simulink model "multirotor_gn_model"  (R2025b)
settings: Solver=ode3  StartTime=0.0  StopTime=600  FixedStep=simulationSampleTime  RelTol=1e-3
values from neighbouring files (symbols this model uses):
  guidanceParams = [cfg.guidance.acceptanceRadiusM;      cfg.flight.transitSpeedMps; cfg.flight.searchSpeedMps;      cfg.flight.climbSpeedMps; cfg.flight.descentSpeedMps;      cfg.guidance.slowdownRadiusM;      cfg.guidance.landingHorizontalToleranceM;      cfg.guidance.landingAltitudeToleranceM]    [run_multirotor_mission.m]
  navigationFilterCoefficient = cfg.navigation.filterCoefficient    [run_multirotor_mission.m]
  navigationNoiseSeeds = mod(round(cfg.randomSeed)+(1:3)'*997,2^31-1)    [run_multirotor_mission.m]
  navigationNoiseVariance = cfg.navigation.positionNoiseStdM^2    [run_multirotor_mission.m]
  routeCount = mission.routeCount    [run_multirotor_mission.m]
  routePhasePadded = zeros(cfg.simulation.maxWaypoints,1)    [run_multirotor_mission.m]
  routeWaypointsPadded = zeros(cfg.simulation.maxWaypoints,3)    [run_multirotor_mission.m]
  simulationSampleTime = cfg.simulation.sampleTimeSec    [run_multirotor_mission.m]
  vehicleTimeConstantSec = cfg.vehicle.velocityTimeConstantSec    [run_multirotor_mission.m]
libraries: simulink x1
settings Model: Creator=andrei  LastModifiedBy=andrei
settings DataIOCC: SignalLogging=off

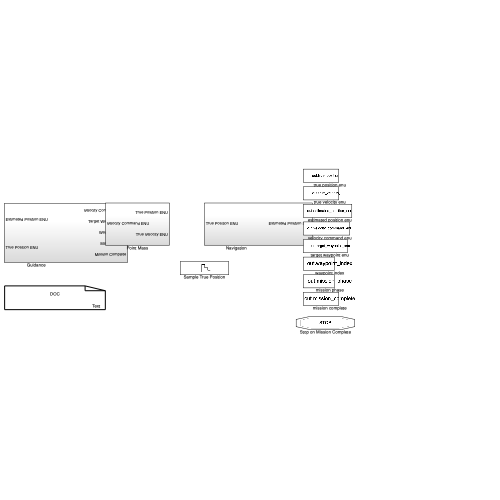
[thumbnail: Simulink's stored preview of the top-level diagram]
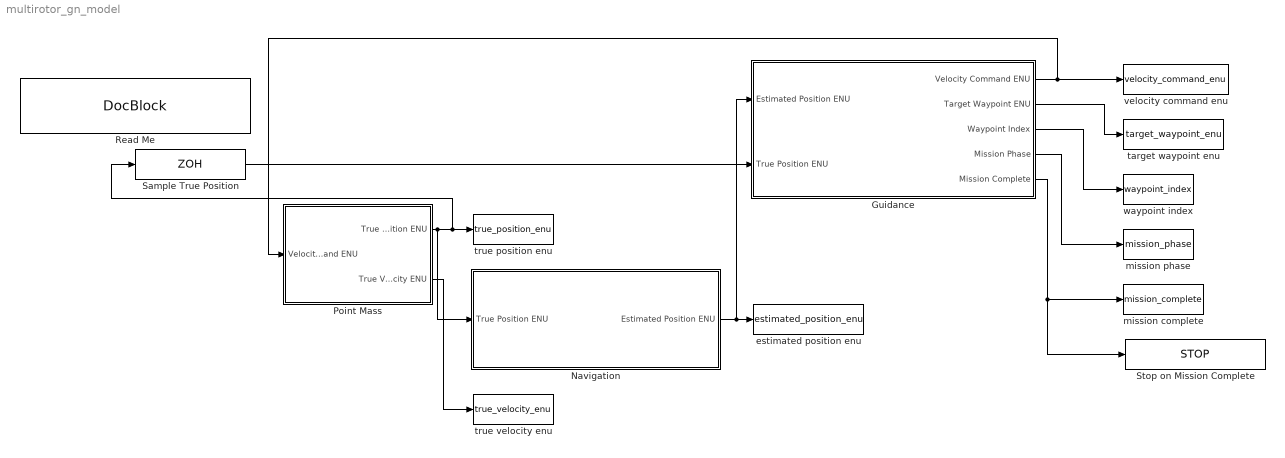
== system multirotor_gn_model ==
  Guidance : Subsystem
  Navigation : Subsystem
  Point Mass : Subsystem
  Read Me : simulink/Model-Wide Utilities/DocBlock  DocumentType=Text
  Sample True Position : ZeroOrderHold  SampleTime=simulationSampleTime
  Stop on Mission Complete : Stop
  estimated position enu : ToWorkspace  VariableName=estimated_position_enu  SaveFormat=Timeseries  SampleTime=-1
  mission complete : ToWorkspace  VariableName=mission_complete  SaveFormat=Timeseries  SampleTime=-1
  mission phase : ToWorkspace  VariableName=mission_phase  SaveFormat=Timeseries  SampleTime=-1
  target waypoint enu : ToWorkspace  VariableName=target_waypoint_enu  SaveFormat=Timeseries  SampleTime=-1
  true position enu : ToWorkspace  VariableName=true_position_enu  SaveFormat=Timeseries  SampleTime=-1
  true velocity enu : ToWorkspace  VariableName=true_velocity_enu  SaveFormat=Timeseries  SampleTime=-1
  velocity command enu : ToWorkspace  VariableName=velocity_command_enu  SaveFormat=Timeseries  SampleTime=-1
  waypoint index : ToWorkspace  VariableName=waypoint_index  SaveFormat=Timeseries  SampleTime=-1
  wires:
  Guidance/5(Mission Complete) -> Stop on Mission Complete/1, mission complete/1
  Guidance/4(Mission Phase) -> mission phase/1
  Guidance/2(Target Waypoint ENU) -> target waypoint enu/1
  Guidance/1(Velocity Command ENU) -> velocity command enu/1, Point Mass/1(Velocity Command ENU)
  Navigation/1(Estimated Position ENU) -> estimated position enu/1, Guidance/1(Estimated Position ENU)
  Point Mass/2(True Velocity ENU) -> true velocity enu/1
  Guidance/3(Waypoint Index) -> waypoint index/1
  Point Mass/1(True Position ENU) -> true position enu/1, Sample True Position/1, Navigation/1(True Position ENU)
  Sample True Position/1 -> Guidance/2(True Position ENU)

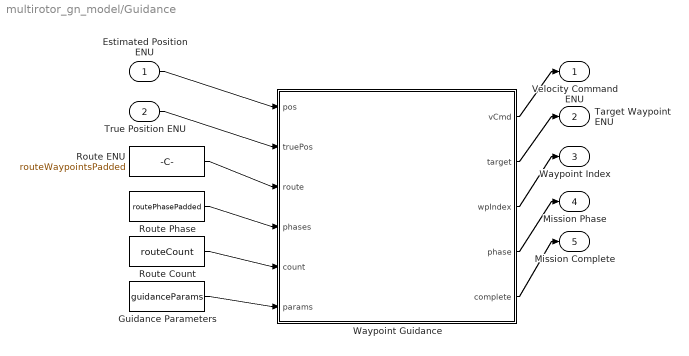
== system multirotor_gn_model/Guidance ==
  Estimated Position ENU : Inport  PortDimensions=3
  True Position ENU : Inport  Port=2  PortDimensions=3
  Guidance Parameters : Constant  Value=guidanceParams
  Route Count : Constant  Value=routeCount
  Route ENU : Constant  Value=routeWaypointsPadded
  Route Phase : Constant  Value=routePhasePadded
  Waypoint Guidance : MATLAB Function  TreatAsAtomicUnit=on
  Velocity Command ENU : Outport
  Target Waypoint ENU : Outport  Port=2
  Waypoint Index : Outport  Port=3
  Mission Phase : Outport  Port=4
  Mission Complete : Outport  Port=5
  wires:
  Estimated Position ENU/1 -> Waypoint Guidance/1(pos)
  True Position ENU/1 -> Waypoint Guidance/2(truePos)
  Route ENU/1 -> Waypoint Guidance/3(route)
  Route Phase/1 -> Waypoint Guidance/4(phases)
  Route Count/1 -> Waypoint Guidance/5(count)
  Guidance Parameters/1 -> Waypoint Guidance/6(params)
  Waypoint Guidance/1(vCmd) -> Velocity Command ENU/1
  Waypoint Guidance/2(target) -> Target Waypoint ENU/1
  Waypoint Guidance/3(wpIndex) -> Waypoint Index/1
  Waypoint Guidance/4(phase) -> Mission Phase/1
  Waypoint Guidance/5(complete) -> Mission Complete/1

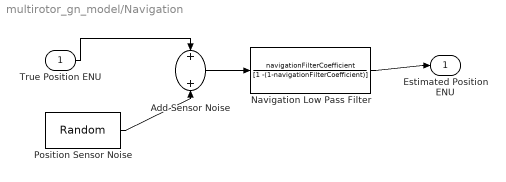
== system multirotor_gn_model/Navigation ==
  True Position ENU : Inport  PortDimensions=3
  Add Sensor Noise : Sum
  Navigation Low Pass Filter : DiscreteFilter  Numerator=navigationFilterCoefficient  Denominator=[1 -(1-navigationFilterCoefficient)]  SampleTime=simulationSampleTime
  Position Sensor Noise : RandomNumber  Mean=[0;0;0]  Variance=navigationNoiseVariance*[1;1;1]  Seed=navigationNoiseSeeds  SampleTime=simulationSampleTime
  Estimated Position ENU : Outport
  wires:
  True Position ENU/1 -> Add Sensor Noise/1
  Position Sensor Noise/1 -> Add Sensor Noise/2
  Add Sensor Noise/1 -> Navigation Low Pass Filter/1
  Navigation Low Pass Filter/1 -> Estimated Position ENU/1

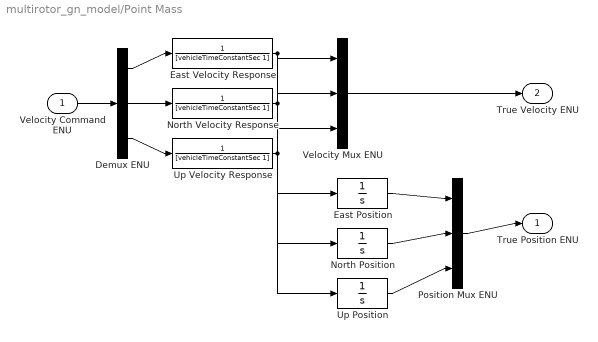
== system multirotor_gn_model/Point Mass ==
  Velocity Command ENU : Inport  PortDimensions=3
  Demux ENU : Demux  Outputs=3
  East Position : Integrator
  East Velocity Response : TransferFcn  Numerator=1  Denominator=[vehicleTimeConstantSec 1]
  North Position : Integrator
  North Velocity Response : TransferFcn  Numerator=1  Denominator=[vehicleTimeConstantSec 1]
  Position Mux ENU : Mux  Inputs=3
  Up Position : Integrator  LimitOutput=on  LowerSaturationLimit=0
  Up Velocity Response : TransferFcn  Numerator=1  Denominator=[vehicleTimeConstantSec 1]
  Velocity Mux ENU : Mux  Inputs=3
  True Position ENU : Outport
  True Velocity ENU : Outport  Port=2
  wires:
  Demux ENU/1 -> East Velocity Response/1
  Demux ENU/2 -> North Velocity Response/1
  Demux ENU/3 -> Up Velocity Response/1
  East Velocity Response/1 -> Velocity Mux ENU/1, East Position/1
  East Position/1 -> Position Mux ENU/1
  North Velocity Response/1 -> Velocity Mux ENU/2, North Position/1
  North Position/1 -> Position Mux ENU/2
  Up Velocity Response/1 -> Velocity Mux ENU/3, Up Position/1
  Up Position/1 -> Position Mux ENU/3
  Velocity Command ENU/1 -> Demux ENU/1
  Position Mux ENU/1 -> True Position ENU/1
  Velocity Mux ENU/1 -> True Velocity ENU/1

== matlab function multirotor_gn_model/Guidance/Waypoint Guidance ==
  data: pos input; vCmd output; truePos input; route input; phases input; count input; params input; target output; wpIndex output; phase output; complete output
function [vCmd,target,wpIndex,phase,complete] = fcn(pos,truePos,route,phases,count,params)
%#codegen
[vCmd,target,wpIndex,phase,complete] = guidance_step(pos,truePos,route,phases,count,params);
end
